simulink model "boost_pid"  (R2025a)
settings: Solver=FixedStepAuto  StartTime=0.0  StopTime=T_sim  FixedStep=Ts_pwr  RelTol=1e-3
values from neighbouring files (symbols this model uses):
  C = 220e-6    (= 0.00022)    [param_boost_pblb.m]
  D_max = 0.85    [param_boost_pblb.m]
  D_min = 0    [param_boost_pblb.m]
  Kb = Kb0    (= 4000)    [param_boost_pblb.m]
  Kd = Kd0    (= 6.6e-06)    [param_boost_pblb.m]    (also in tuning_pid.m = Kd0; uji_skenario.m = 2*Kd0)
  Ki = Ki0    (= 6.1)    [param_boost_pblb.m]    (also in tuning_pid.m = Ki0; uji_skenario.m = Ki0)
  Kp = Kp0    (= 0.0014)    [param_boost_pblb.m]    (also in tuning_pid.m = Kp0; uji_skenario.m = Kp0)
  L = 680e-6    (= 0.00068)    [param_boost_pblb.m]
  N = N0    (= 10000)    [param_boost_pblb.m]
  R_nom = 32    [param_boost_pblb.m]    (also in uji_skenario.m)
  Ts_ctrl = 1/fsw    (= 5e-05)    [param_boost_pblb.m]
  Ts_pwr = 5e-7    (= 5e-07)    [param_boost_pblb.m]    (also in tuning_pid.m; uji_skenario.m = 2e-07)
  Vin_nom = 24    [param_boost_pblb.m]    (also in uji_skenario.m)
  Vref = 48    [param_boost_pblb.m]
libraries: spsGroundLib x3, spsSeriesRLCBranchLib x3, spsCurrentMeasurementLib x2, spsDCVoltageSourceLib x1, spsDiodeLib x1, spsMosfetLib x1, slpidlib x1, spsPWMGeneratorDCDCLib x1, spsVoltageMeasurementLib x1, sps_lib x1
settings Model: Creator=first  LastModifiedBy=first
settings DataIOCC: SignalLogging=off

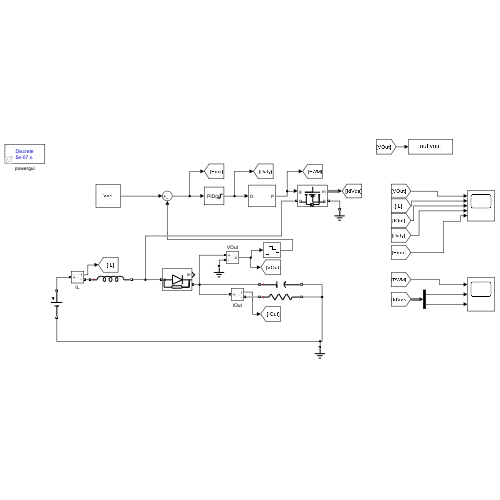
[thumbnail: Simulink's stored preview of the top-level diagram]
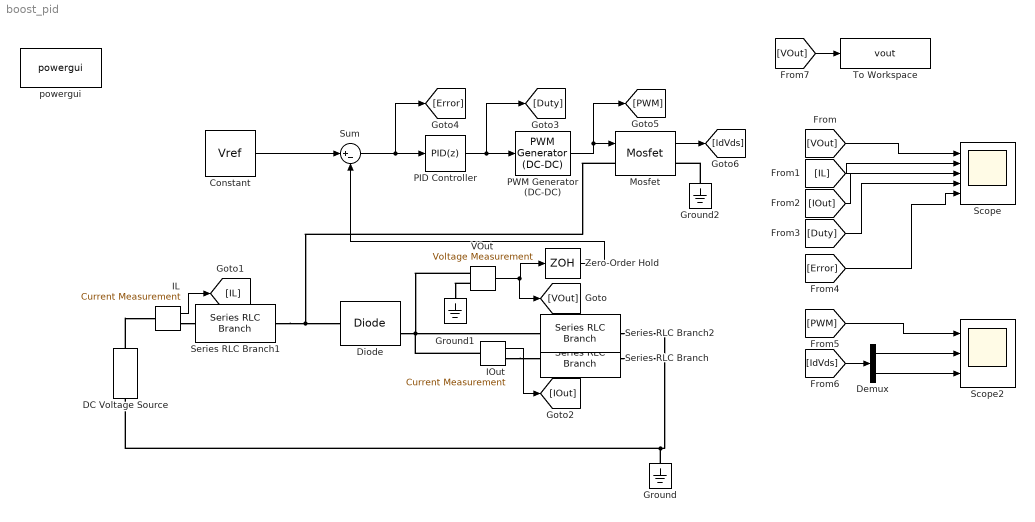
== system boost_pid ==
  Constant : Constant  Value=Vref
  DC Voltage Source : spsDCVoltageSourceLib/DC Voltage Source  Amplitude=Vin_nom  Measurements=None
  Demux : Demux  Outputs=2
  Diode : spsDiodeLib/Diode  Ron=Ron_D  Lon=0  Vf=Vf_D  IC=0  UseSnubber=0  Rs=1e5  Cs=inf  Measurements=on
  Ground : spsGroundLib/Ground  LConnTagsString=a
  Ground1 : spsGroundLib/Ground  LConnTagsString=a
  Ground2 : spsGroundLib/Ground  LConnTagsString=a
  IL : spsCurrentMeasurementLib/Current Measurement  PhasorSimulation=off  OutputType=Complex  PSBequivalent=0
  IOut : spsCurrentMeasurementLib/Current Measurement  PhasorSimulation=off  OutputType=Complex  PSBequivalent=0
  Mosfet : spsMosfetLib/Mosfet  Ron=Ron_Q  Lon=0  Rd=0.01  Vfd=0  IC=0  Rs=1e5  Cs=inf  Measurements=on
  PID Controller : slpidlib/PID Controller  Controller=PID  Form=Parallel  TimeDomain=Discrete-time  UseExternalTs=off  SampleTime=Ts_ctrl  IntegratorMethod=Forward Euler  FilterMethod=Forward Euler  ControllerParametersSource=internal  P=Kp  I=Ki  UseKiTs=off  D=Kd  UseExternalDerivativeSource=off  N=N  UseFilter=on  TunerSelectOption=Transfer Function Based (PID Tuner App)  InitialConditionSource=internal  InitialConditionForIntegrator=0  InitialConditionForFilter=0  DifferentiatorICPrevScaledInput=0  ExternalReset=none  TrackingMode=off  Kt=1  LimitOutput=on  SatLimitsSource=internal  UpperSaturationLimit=D_max  LowerSaturationLimit=D_min  LinearizeAsGain=on  AntiWindupMode=back-calculation  Kb=Kb  LimitIntegrator=off  UpperIntegratorSaturationLimit=inf  LowerIntegratorSaturationLimit=-inf  POutMin=[]  POutMax=[]  IOutMin=[]  IOutMax=[]  DOutMin=[]  DOutMax=[]  NOutMin=[]  NOutMax=[]  SumOutMin=[]  SumOutMax=[]  SaturationOutMin=[]  SaturationOutMax=[]  PParamMin=[]  PParamMax=[]  IParamMin=[]  IParamMax=[]  DParamMin=[]  DParamMax=[]  NParamMin=[]  NParamMax=[]  KbParamMin=[]  KbParamMax=[]  KtParamMin=[]  KtParamMax=[]  KbOutMin=[]  KbOutMax=[]  KtOutMin=[]  KtOutMax=[]  IntegratorOutMin=[]  IntegratorOutMax=[]  FilterOutMin=[]  FilterOutMax=[]  SumI1OutMin=[]  SumI1OutMax=[]  SumI2OutMin=[]  SumI2OutMax=[]  SumI3OutMin=[]  SumI3OutMax=[]  SumI4OutMin=[]  SumI4OutMax=[]  SumDOutMin=[]  SumDOutMax=[]  DifferentiatorOutMin=[]  DifferentiatorOutMax=[]  FilterDiffOutCoefMin=[]  FilterDiffOutCoefMax=[]  ReciprocalOutMin=[]  ReciprocalOutMax=[]  SumDenOutMin=[]  SumDenOutMax=[]  SumNumOutMin=[]  SumNumOutMax=[]  DivideOutMin=[]  DivideOutMax=[]  UdiffTsProdOutMin=[]  UdiffTsProdOutMax=[]  NTsProdOutMin=[]  NTsProdOutMax=[]  UintegralTsProdOutMin=[]  UintegralTsProdOutMax=[]  UngainTsProdOutMin=[]  UngainTsProdOutMax=[]  ClampingZeroOutDataTypeStr=Inherit: Inherit via back propagation  ClampingZeroOutMin=[]  ClampingZeroOutMax=[]  FilterDenConstantOutDataTypeStr=Inherit: Inherit via back propagation  FilterDenConstantOutMin=[]  FilterDenConstantOutMax=[]  PCopyOutDataTypeStr=Inherit: Inherit via back propagation  PCopyOutMin=[]  PCopyOutMax=[]  NCopyOutDataTypeStr=Inherit: Inherit via back propagation  NCopyOutMin=[]  NCopyOutMax=[]  IntegratorContinuousStateAttributes=''  IntegratorStateMustResolveToSignalObject=off  IntegratorRTWStateStorageClass=Auto  FilterContinuousStateAttributes=''  FilterStateMustResolveToSignalObject=off  FilterRTWStateStorageClass=Auto  ParallelPVariant=InternalParameters  IdealPVariant=Disabled  IVariant=InternalParameters  DVariant=InternalParameters  IntegratorVariant=Discrete  SatVariant=Enabled  AWVariant=BackCalculation  PCopyVariant=Disabled  TRVariant=Disabled  FdbkBlocksVariant=Forward  IdealPFdbkVariant=Disabled  SatFdbkVariant=Disabled  DerivativeFilterVariant=ForwardEulerFilter  NVariant=InternalParameters  NCopyVariant=Disabled  FilterICVariant=InternalICsFilter  IntegratorICVariant=InternalICs  ExternalResetVariant=Disabled  TRSumVariant=Passthrough  SumFdbkVariant=Disabled  SumVariant=Sum_PID  TsampFilterVariant=InternalTs  TsampNgainVariant=Passthrough  TsampIntegralVariant=Disabled_SignalSpec  ExternalSaturationOutDataTypeStr=Inherit: Same as second input  DerivativeSourceVariant=ErrorSignal  PreIntVariant=InternalPreInt
  PWM Generator (DC-DC) : spsPWMGeneratorDCDCLib/PWM Generator (DC-DC)  Fsw=fsw  Ts=0
  Scope : Scope  NumInputPorts=5
      settings: ActiveDisplayYMinimum=-1  ActiveDisplayYMaximum=1  DataLoggingDecimation=10
  Scope2 : Scope  NumInputPorts=3
      settings: ActiveDisplayYMinimum=-0.8  ActiveDisplayYMaximum=70  DataLoggingDecimation=10  DataLoggingVariableName=ScopeData2
  Series RLC Branch : spsSeriesRLCBranchLib/Series RLC Branch  LConnTagsString=__new0  RConnTagsString=__new0  BranchType=R  Resistance=R_nom  Inductance=1e-3  SetiL0=off  InitialCurrent=0  Capacitance=1e-6  Setx0=off  InitialVoltage=0  Measurements=None
  Series RLC Branch1 : spsSeriesRLCBranchLib/Series RLC Branch  LConnTagsString=__new0  RConnTagsString=__new0  BranchType=L  Resistance=1  Inductance=L  SetiL0=off  InitialCurrent=0  Capacitance=1e-6  Setx0=off  InitialVoltage=0  Measurements=None
  Series RLC Branch2 : spsSeriesRLCBranchLib/Series RLC Branch  LConnTagsString=__new0  RConnTagsString=__new0  BranchType=C  Resistance=1  Inductance=1e-3  SetiL0=off  InitialCurrent=0  Capacitance=C  Setx0=on  InitialVoltage=Vc0  Measurements=None
  Sum : Sum  Inputs=|+-
  To Workspace : ToWorkspace  VariableName=vout  SaveFormat=Timeseries  SampleTime=-1
  VOut : spsVoltageMeasurementLib/Voltage Measurement  PhasorSimulation=off  OutputType=Complex  PSBequivalent=0
  Zero-Order Hold : ZeroOrderHold  SampleTime=Ts_ctrl
  powergui : sps_lib/powergui  Priority=1  SimulationMode=Discrete  SampleTime=Ts_pwr  frequency=60  Iterations=50  frequencyindice=0  Pbase=100e6  ErrMax=1e-4  UnitsV=kV  UnitsW=MW  buscounter=0  FunctionMessages=off  echomessages=off  EnableUseOfTLC=off  CurrentSourceSwitches=off  DisableSnubberDevices=off  DisableRonSwitches=off  DisableVfSwitches=off  DisplayEquations=off  AutomaticDiscreteSolvers=off  SolverType=Tustin/Backward Euler (TBE)  Interpol=off  ExternalGateDelay=off  methode=off  Ts=100  x0status=blocks  SPID=on  SwTol=0  HookPort=off  NonlinearTolerance=1e-4  nMaxIteration=100  ContinueOnMaxIteration=off  RestoreLinks=warning  ResistiveCurrentMeasurement=off  Frange=[0:2:500]  Ylog=off  Xlog=on  ShowGrid=off  save=off  variable=ZData  structure=0  ZoomFFT=off  StartTime=0.0  cycles=1  DisplayStyle=1  fundamental=60  FreqAxis=off  MaxFrequency=1000  frequencyindicesteady=1  RmsSteady=1  display=off
  wires:
  VOut/1 -> [VOut], Zero-Order Hold/1
  Constant/1 -> Sum/1
  Zero-Order Hold/1 -> Sum/2
  Sum/1 -> [Error], PID Controller/1
  PID Controller/1 -> [Duty], PWM Generator (DC-DC)/1
  PWM Generator (DC-DC)/1 -> [PWM], Mosfet/1
  [VOut] -> Scope/1
  IL/1 -> [IL]
  [IL] -> Scope/2
  IOut/1 -> [IOut]
  [IOut] -> Scope/3
  [Duty] -> Scope/4
  [Error] -> Scope/5
  [PWM] -> Scope2/1
  Demux/1 -> Scope2/2
  Demux/2 -> Scope2/3
  Mosfet/1 -> [IdVds]
  [IdVds] -> Demux/1
  [VOut] -> To Workspace/1
  connections:
  Series RLC Branch1/RConn1 -- Mosfet/LConn1 -- Diode/LConn1
  Ground/LConn1 -- DC Voltage Source/LConn1 -- Series RLC Branch/RConn1 -- Series RLC Branch2/RConn1
  VOut/LConn2 -- Ground1/LConn1
  IL/RConn1 -- Series RLC Branch1/LConn1
  DC Voltage Source/RConn1 -- IL/LConn1
  IOut/RConn1 -- Series RLC Branch/LConn1
  Diode/RConn1 -- VOut/LConn1 -- IOut/LConn1 -- Series RLC Branch2/LConn1
  Ground2/LConn1 -- Mosfet/RConn1
